simulink model "sm_Experimental_Setup"  (R2020b)
settings: Solver=VariableStepAuto  StartTime=0.0  StopTime=2000  RelTol=1e-3
values from neighbouring files (symbols this model uses):
  ACCEPTABLE_DELTA = 0.05    [code_DDPG_Training.m]    (also in code_Experimental_Setup.m; code_SA_TF_Estimator.m)
  fD = 3.5243/2    (= 1.76215)    [code_DDPG_Training.m]    (also in code_Experimental_Setup.m; code_SA_TF_Estimator.m = 3.5243)
  fS = 8.4000/2    (= 4.2)    [code_DDPG_Training.m]    (also in code_Experimental_Setup.m; code_SA_TF_Estimator.m = 8.4)
  TIME_DELAY = 2.5/2    (= 1.25)    [code_DDPG_Training.m]    (also in code_Experimental_Setup.m; code_SA_TF_Estimator.m = 2.5)
  Ts = 1.0    (= 1)    [code_DDPG_Training.m]    (also in code_Experimental_Setup.m; code_SA_TF_Estimator.m)
undefined symbols (not defined in the file or in its folder): DiscIntNeverNeededParam, sigbuilder_block
libraries: simulink x2, pid_lib x1, rllib x1
settings Model: Creator=rajeshs  LastModifiedBy=rajeshs
settings SFSimCC: CustomCodeUndefinedFunction=UseInterfaceOnly

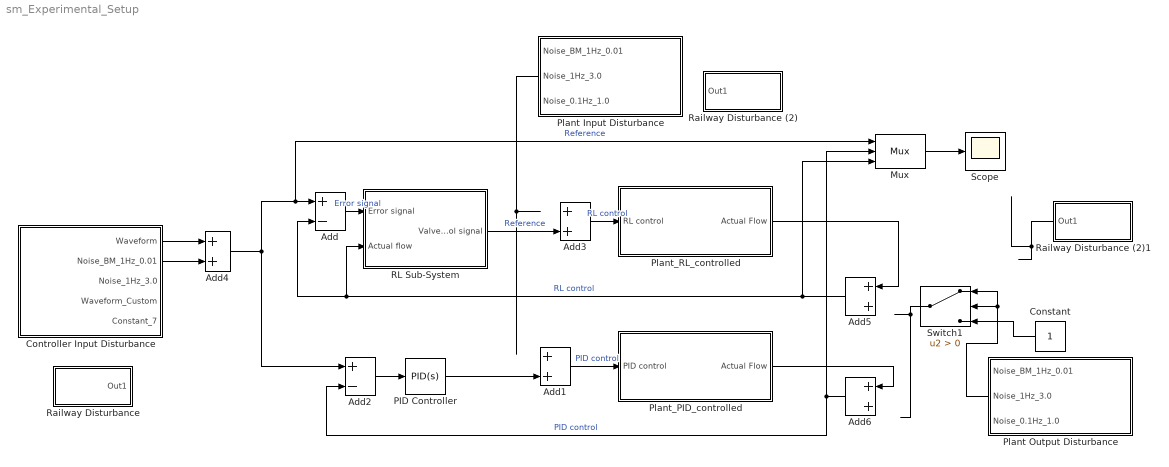
== system sm_Experimental_Setup ==
  Add : Sum  Inputs=+-
  Add{1,3..6} (5 alike) : Sum
  Add2 : Sum  Inputs=+-
  Constant : Constant
  Controller Input Disturbance : Subsystem  Tag=STV Subsys  LoadFcn=sigbuilder_block('load');  StartFcn=sigbuilder_block('start');  StopFcn=sigbuilder_block('stop');  ClipboardFcn=sigbuilder_block('clipboard');  mask(Sigbuilder block){tuvar=[0:10]}
      mask help: Simulink:masks:SigbuilderBlock_MD
      mask init:
      | if ~strcmp(get_param(bdroot(gcbh),'SimulationStatus'),'stopped') tuvar = sigbuilder_block('maskInit'); end
      settings: CopyFcn=sigbuilder_block('copy');  DeleteFcn=sigbuilder_block('delete');  ModelCloseFcn=sigbuilder_block('modelClose');  PreSaveFcn=sigbuilder_block('preSave');  PauseFcn=sigbuilder_block('pause');  ContinueFcn=sigbuilder_block('continue');  NameChangeFcn=sigbuilder_block('namechange');  OpenFcn=sigbuilder_block('open',[329.25 -26.25 324 449.25 ]);  CloseFcn=sigbuilder_block('close');
      mask Display: plot(0, 0, 100, 100,[2, 2, 32, 32, 2], [68, 8, 8, 68, 68],[32, 2], [38, 38], [32, 19, 2],[53, 60, 44], [32, 17, 17, 2],[16, 16, 31, 31]);txt = getActiveGroup(gcbh);text(2, 100, txt,'verticalAlignment', 'top');
  Mux : Mux  Inputs=3
      settings: DisplayOption=signals
  PID Controller : pid_lib/PID Controller  Controller=PID  Form=Parallel  TimeDomain=Continuous-time  UseExternalTs=off  SampleTime=-1  IntegratorMethod=Forward Euler  FilterMethod=Forward Euler  ControllerParametersSource=internal  P=0.3631  I=0.0045  D=-1.7202  UseFilter=on  N=0.0114  TunerSelectOption=Transfer Function Based (PID Tuner App)  InitialConditionSource=internal  InitialConditionForIntegrator=0  InitialConditionForFilter=0  DifferentiatorICPrevScaledInput=0  ExternalReset=none  TrackingMode=off  Kt=1  LimitOutput=off  SatLimitsSource=internal  UpperSaturationLimit=inf  LowerSaturationLimit=-inf  LinearizeAsGain=on  AntiWindupMode=none  Kb=1  POutMin=[]  POutMax=[]  IOutMin=[]  IOutMax=[]  DOutMin=[]  DOutMax=[]  NOutMin=[]  NOutMax=[]  SumOutMin=[]  SumOutMax=[]  SaturationOutMin=[]  SaturationOutMax=[]  PParamMin=[]  PParamMax=[]  IParamMin=[]  IParamMax=[]  DParamMin=[]  DParamMax=[]  NParamMin=[]  NParamMax=[]  KbParamMin=[]  KbParamMax=[]  KtParamMin=[]  KtParamMax=[]  KbOutMin=[]  KbOutMax=[]  KtOutMin=[]  KtOutMax=[]  IntegratorOutMin=[]  IntegratorOutMax=[]  FilterOutMin=[]  FilterOutMax=[]  SumI1OutMin=[]  SumI1OutMax=[]  SumI2OutMin=[]  SumI2OutMax=[]  SumI3OutMin=[]  SumI3OutMax=[]  SumI4OutMin=[]  SumI4OutMax=[]  SumDOutMin=[]  SumDOutMax=[]  DifferentiatorOutMin=[]  DifferentiatorOutMax=[]  FilterDiffOutCoefMin=[]  FilterDiffOutCoefMax=[]  ReciprocalOutMin=[]  ReciprocalOutMax=[]  SumDenOutMin=[]  SumDenOutMax=[]  SumNumOutMin=[]  SumNumOutMax=[]  DivideOutMin=[]  DivideOutMax=[]  UdiffTsProdOutMin=[]  UdiffTsProdOutMax=[]  NTsProdOutMin=[]  NTsProdOutMax=[]  UintegralTsProdOutMin=[]  UintegralTsProdOutMax=[]  UngainTsProdOutMin=[]  UngainTsProdOutMax=[]  IntegratorContinuousStateAttributes=''  IntegratorStateMustResolveToSignalObject=off  IntegratorRTWStateStorageClass=Auto  FilterContinuousStateAttributes=''  FilterStateMustResolveToSignalObject=off  FilterRTWStateStorageClass=Auto  ParallelPVariant=InternalParameters  IdealPVariant=Disabled  IVariant=InternalParameters  DVariant=InternalParameters  IntegratorVariant=Continuous  SatVariant=Disabled  AWVariant=Passthrough  PCopyVariant=Disabled  TRVariant=Disabled  FdbkBlocksVariant=Forward  IdealPFdbkVariant=Disabled  SatFdbkVariant=Disabled  DerivativeFilterVariant=ContFilter  NVariant=InternalParameters  NCopyVariant=Disabled  FilterICVariant=InternalICsFilter  IntegratorICVariant=InternalICs  ExternalResetVariant=Disabled  TRSumVariant=Passthrough  SumFdbkVariant=Disabled  SumVariant=Sum_PID  TsampFilterVariant=InternalTs  TsampNgainVariant=Passthrough  TsampIntegralVariant=Passthrough  ExternalSaturationOutDataTypeStr=Inherit: Same as second input
  Plant Input Disturbance : Subsystem  Tag=STV Subsys  LoadFcn=sigbuilder_block('load');  StartFcn=sigbuilder_block('start');  StopFcn=sigbuilder_block('stop');  ClipboardFcn=sigbuilder_block('clipboard');  mask(Sigbuilder block){tuvar=[0:10]}
      mask help: Simulink:masks:SigbuilderBlock_MD
      mask init:
      | if ~strcmp(get_param(bdroot(gcbh),'SimulationStatus'),'stopped') tuvar = sigbuilder_block('maskInit'); end
      settings: CopyFcn=sigbuilder_block('copy');  DeleteFcn=sigbuilder_block('delete');  ModelCloseFcn=sigbuilder_block('modelClose');  PreSaveFcn=sigbuilder_block('preSave');  PauseFcn=sigbuilder_block('pause');  ContinueFcn=sigbuilder_block('continue');  NameChangeFcn=sigbuilder_block('namechange');  OpenFcn=sigbuilder_block('open',[6 6 1012.5 506.25 ]);  CloseFcn=sigbuilder_block('close');
      mask Display: plot(0, 0, 100, 100,[2, 2, 32, 32, 2], [68, 8, 8, 68, 68],[32, 2], [38, 38], [32, 19, 2],[53, 60, 44], [32, 17, 17, 2],[16, 16, 31, 31]);txt = getActiveGroup(gcbh);text(2, 100, txt,'verticalAlignment', 'top');
  Plant Output Disturbance : Subsystem  Tag=STV Subsys  LoadFcn=sigbuilder_block('load');  StartFcn=sigbuilder_block('start');  StopFcn=sigbuilder_block('stop');  ClipboardFcn=sigbuilder_block('clipboard');  mask(Sigbuilder block){tuvar=[0:10]}
      mask help: Simulink:masks:SigbuilderBlock_MD
      mask init:
      | if ~strcmp(get_param(bdroot(gcbh),'SimulationStatus'),'stopped') tuvar = sigbuilder_block('maskInit'); end
      settings: CopyFcn=sigbuilder_block('copy');  DeleteFcn=sigbuilder_block('delete');  ModelCloseFcn=sigbuilder_block('modelClose');  PreSaveFcn=sigbuilder_block('preSave');  PauseFcn=sigbuilder_block('pause');  ContinueFcn=sigbuilder_block('continue');  NameChangeFcn=sigbuilder_block('namechange');  OpenFcn=sigbuilder_block('open',[6 6 1012.5 506.25 ]);  CloseFcn=sigbuilder_block('close');
      mask Display: plot(0, 0, 100, 100,[2, 2, 32, 32, 2], [68, 8, 8, 68, 68],[32, 2], [38, 38], [32, 19, 2],[53, 60, 44], [32, 17, 17, 2],[16, 16, 31, 31]);txt = getActiveGroup(gcbh);text(2, 100, txt,'verticalAlignment', 'top');
  Plant_PID_controlled : Subsystem
  Plant_RL_controlled : Subsystem
  RL Sub-System : Subsystem
  Railway Disturbance : Subsystem
  Railway Disturbance (2) : Subsystem
  Railway Disturbance (2)1 : Subsystem
  Scope : Scope
  Switch1 : Switch  Criteria=u2 > Threshold
  wires:
  Add/1 -> RL Sub-System/1(Error signal)  "Error signal"
  Add5/1 -> Mux/3, Add/2, RL Sub-System/2(Actual flow)  "RL control"
  PID Controller/1 -> Add1/2
  Add2/1 -> PID Controller/1
  Mux/1 -> Scope/1
  Add1/1 -> Plant_PID_controlled/1(PID control)  "PID control"
  Controller Input Disturbance/1(Waveform) -> Add4/1
  Add6/1 -> Mux/2, Add2/2  "PID control"
  Constant/1 -> Switch1/3
  Railway Disturbance (2)1/1(Out1) -> ?
  Switch1/1 -> ?
  Plant Input Disturbance/2(Noise_1Hz_3.0) -> ?
  Add3/1 -> Plant_RL_controlled/1(RL control)  "RL control"
  Plant_RL_controlled/1(Actual Flow) -> Add5/1
  Plant_PID_controlled/1(Actual Flow) -> Add6/1
  Controller Input Disturbance/2(Noise_BM_1Hz_0.01) -> Add4/2
  Add4/1 -> Add2/1, Mux/1, Add/1  "Reference"
  RL Sub-System/1(Valve control signal) -> Add3/2  "Reference"
  Plant Output Disturbance/2(Noise_1Hz_3.0) -> Switch1/2, Switch1/1

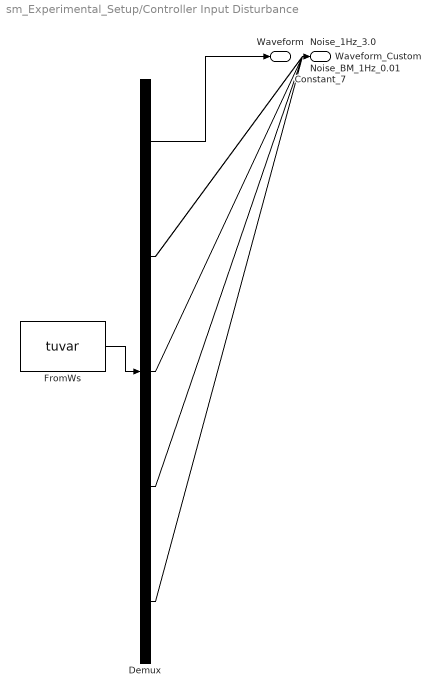
== system sm_Experimental_Setup/Controller Input Disturbance ==
  Demux : Demux  Tag=STV Demux  Outputs=5
      settings: DisplayOption=none
  FromWs : FromWorkspace  Tag=STV FromWs  VariableName=tuvar
      SigBuilderData=|
      | common.afterFinalStr = 'Extrapolate'
      | common.sampleTime = 0
      | dataSet.timeRange = [0 2000]
      | dataSet.name = 'Signals'
      | sbobj.Groups.Name = 'Signals'
      | sbobj.Groups.Signals(1).Name = 'Waveform'
      | sbobj.Groups.Signals(1).XData = [0 752 752 1500 1500 1750 1750 2000]
      | sbobj.Groups.Signals(1).YData = [100 100 25 25 75 75 25 25]
      | sbobj.Groups.Signals(2).Name = 'Noise_BM_1Hz_0.01'
      | sbobj.Groups.Signals(2).XData = [0 1 2 3 4 5 6 7 8 9 10 11 ... (2001 elements, 1x2001)]
      | sbobj.Groups.Signals(2).YData = [0.0109017282673 -0.00358703225346 -0.0012992763049 0.00733737523776 0.00120331570317 0.0113633128469 -0.00686773118719 0.00471682863443 0.00288342465456 0.0139185483505 -0.0134550201016 7.47406191734e-06 ... (2001 elements, 1x2001)]
      | sbobj.Groups.Signals(3).Name = 'Noise_1Hz_3.0'
      | sbobj.Groups.Signals(3).XData = [0 1 2 3 4 5 6 7 8 9 10 11 ... (2001 elements, 1x2001)]
      | sbobj.Groups.Signals(3).YData = [-1.22103016093 -2.32126408989 6.42034479721 -4.13028289214 0.366124868815 1.68201285192 -3.06458126709 -0.0302582378605 -4.3152453304 1.33545254952 0.451492702689 0.846422939597 ... (2001 elements, 1x2001)]
      | sbobj.Groups.Signals(4).Name = 'Waveform_Custom'
      | sbobj.Groups.Signals(4).XData = [0 100 110 200 290 398 500 600 1000 1050 1225 1400 1500 2000]
      | sbobj.Groups.Signals(4).YData = [75 75 100 100 100 20 20 75 75 10 10 100 100 5]
      | sbobj.Groups.Signals(5).Name = 'Constant_7'
      | sbobj.Groups.Signals(5).XData = [0 2000]
      | sbobj.Groups.Signals(5).YData = [100 100]
      | sbobj.Groups.TimeRange = [0 2000]
  Waveform : Outport  Tag=STV Outport  VectorParamsAs1DForOutWhenUnconnected=off
  Noise_BM_1Hz_0.01 : Outport  Tag=STV Outport  Port=2  VectorParamsAs1DForOutWhenUnconnected=off
  Noise_1Hz_3.0 : Outport  Tag=STV Outport  Port=3  VectorParamsAs1DForOutWhenUnconnected=off
  Waveform_Custom : Outport  Tag=STV Outport  Port=4  VectorParamsAs1DForOutWhenUnconnected=off
  Constant_7 : Outport  Tag=STV Outport  Port=5  VectorParamsAs1DForOutWhenUnconnected=off
  wires:
  Demux/1 -> Waveform/1
  FromWs/1 -> Demux/1
  Demux/2 -> Noise_BM_1Hz_0.01/1
  Demux/3 -> Noise_1Hz_3.0/1
  Demux/4 -> Waveform_Custom/1
  Demux/5 -> Constant_7/1

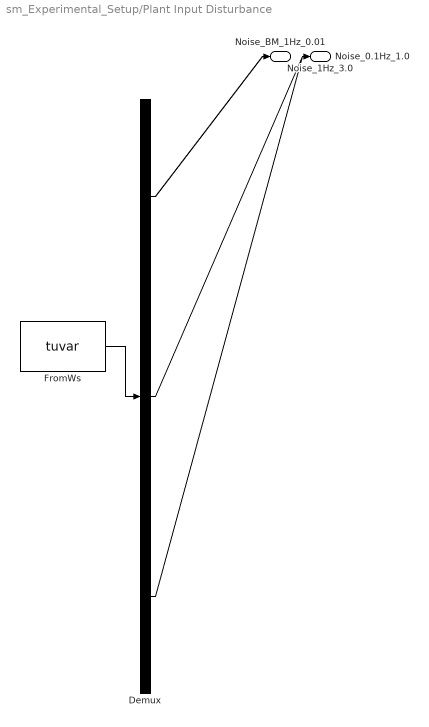
== system sm_Experimental_Setup/Plant Input Disturbance ==
  Demux : Demux  Tag=STV Demux  Outputs=3
      settings: DisplayOption=none
  FromWs : FromWorkspace  Tag=STV FromWs  VariableName=tuvar
      SigBuilderData=|
      | common.afterFinalStr = 'Extrapolate'
      | common.sampleTime = 0
      | dataSet.timeRange = [0 2000]
      | dataSet.name = 'Signals'
      | sbobj.Groups.Name = 'Signals'
      | sbobj.Groups.Signals(1).Name = 'Noise_BM_1Hz_0.01'
      | sbobj.Groups.Signals(1).XData = [0 1 2 3 4 5 6 7 8 9 10 11 ... (2001 elements, 1x2001)]
      | sbobj.Groups.Signals(1).YData = [0.0109017282673 -0.00358703225346 -0.0012992763049 0.00733737523776 0.00120331570317 0.0113633128469 -0.00686773118719 0.00471682863443 0.00288342465456 0.0139185483505 -0.0134550201016 7.47406191734e-06 ... (2001 elements, 1x2001)]
      | sbobj.Groups.Signals(2).Name = 'Noise_1Hz_3.0'
      | sbobj.Groups.Signals(2).XData = [0 1 2 3 4 5 6 7 8 9 10 11 ... (2001 elements, 1x2001)]
      | sbobj.Groups.Signals(2).YData = [-1.79047363866 1.41185835628 -7.19725460522 4.95232912088 1.68989140864 0.114208185443 0.567343325217 3.74247314685 -1.90443716599 -1.78570435989 -0.962472411073 -0.747666280685 ... (2001 elements, 1x2001)]
      | sbobj.Groups.Signals(3).Name = 'Noise_0.1Hz_1.0'
      | sbobj.Groups.Signals(3).XData = [0 10 20 30 40 50 60 70 80 90 100 110 120 130 140 150 160 170 180 190 200 210 220 230 240 250 260 270 280 290 300 310 320 330 340 350 360 370 380 390 400 410 420 430 440 450 460 470 480 490 500 510 520 530 540 550 560 570 580 590 600 610 620 630 640 650 660 670 680 690 700 710 720 730 740 750 760 770 780 790 800 810 820 830 840 850 860 870 880 890 900 910 920 930 940 950 960 970 980 990 1000 1010 1020 1030 1040 1050 1060 1070 1080 1090 1100 1110 1120 1130 1140 1150 1160 1170 1180 1190 1200 1210 1220 1230 1240 1250 1260 1270 1280 1290 1300 1310 1320 1330 1340 1350 1360 1370 1380 1390 1400 1410 1420 1430 1440 1450 1460 1470 1480 1490 1500 1510 1520 1530 1540 1550 1560 1570 1580 1590 1600 1610 1620 1630 1640 1650 1660 1670 1680 1690 1700 1710 1720 1730 1740 1750 1760 1770 1780 1790 1800 1810 1820 1830 1840 1850 1860 1870 1880 1890 1900 1910 1920 1930 1940 1950 1960 1970 1980 1990 2000]
      | sbobj.Groups.Signals(3).YData = [-0.897770229062 -1.24409162366 -0.169459534439 0.984418939663 -0.25104223595 -0.783659850186 0.308330648127 0.156728181712 0.673558474636 0.532804033794 2.10675302476 -1.10578974409 ... (201 elements, 1x201)]
      | sbobj.Groups.TimeRange = [0 2000]
  Noise_BM_1Hz_0.01 : Outport  Tag=STV Outport  VectorParamsAs1DForOutWhenUnconnected=off
  Noise_1Hz_3.0 : Outport  Tag=STV Outport  Port=2  VectorParamsAs1DForOutWhenUnconnected=off
  Noise_0.1Hz_1.0 : Outport  Tag=STV Outport  Port=3  VectorParamsAs1DForOutWhenUnconnected=off
  wires:
  FromWs/1 -> Demux/1
  Demux/1 -> Noise_BM_1Hz_0.01/1
  Demux/2 -> Noise_1Hz_3.0/1
  Demux/3 -> Noise_0.1Hz_1.0/1

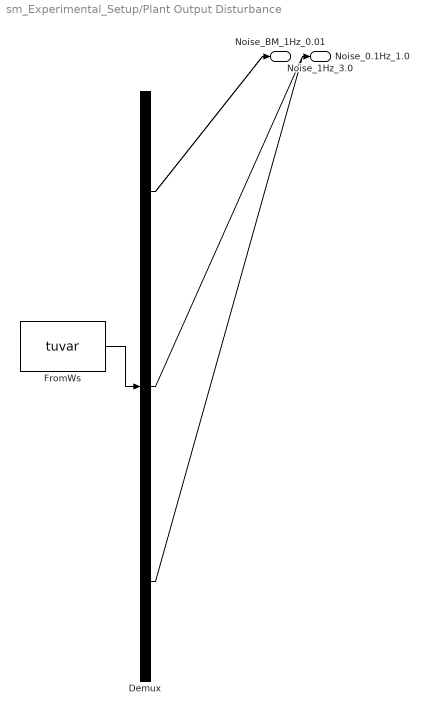
== system sm_Experimental_Setup/Plant Output Disturbance ==
  Demux : Demux  Tag=STV Demux  Outputs=3
      settings: DisplayOption=none
  FromWs : FromWorkspace  Tag=STV FromWs  VariableName=tuvar
      SigBuilderData=|
      | common.afterFinalStr = 'Extrapolate'
      | common.sampleTime = 0
      | dataSet.timeRange = [0 2000]
      | dataSet.name = 'Signals'
      | sbobj.Groups.Name = 'Signals'
      | sbobj.Groups.Signals(1).Name = 'Noise_BM_1Hz_0.01'
      | sbobj.Groups.Signals(1).XData = [0 1 2 3 4 5 6 7 8 9 10 11 ... (2001 elements, 1x2001)]
      | sbobj.Groups.Signals(1).YData = [0.0109017282673 -0.00358703225346 -0.0012992763049 0.00733737523776 0.00120331570317 0.0113633128469 -0.00686773118719 0.00471682863443 0.00288342465456 0.0139185483505 -0.0134550201016 7.47406191734e-06 ... (2001 elements, 1x2001)]
      | sbobj.Groups.Signals(2).Name = 'Noise_1Hz_3.0'
      | sbobj.Groups.Signals(2).XData = [0 1 2 3 4 5 6 7 8 9 10 11 ... (2001 elements, 1x2001)]
      | sbobj.Groups.Signals(2).YData = [-1.22103016093 -2.32126408989 6.42034479721 -4.13028289214 0.366124868815 1.68201285192 -3.06458126709 -0.0302582378605 -4.3152453304 1.33545254952 0.451492702689 0.846422939597 ... (2001 elements, 1x2001)]
      | sbobj.Groups.Signals(3).Name = 'Noise_0.1Hz_1.0'
      | sbobj.Groups.Signals(3).XData = [0 10 20 30 40 50 60 70 80 90 100 110 120 130 140 150 160 170 180 190 200 210 220 230 240 250 260 270 280 290 300 310 320 330 340 350 360 370 380 390 400 410 420 430 440 450 460 470 480 490 500 510 520 530 540 550 560 570 580 590 600 610 620 630 640 650 660 670 680 690 700 710 720 730 740 750 760 770 780 790 800 810 820 830 840 850 860 870 880 890 900 910 920 930 940 950 960 970 980 990 1000 1010 1020 1030 1040 1050 1060 1070 1080 1090 1100 1110 1120 1130 1140 1150 1160 1170 1180 1190 1200 1210 1220 1230 1240 1250 1260 1270 1280 1290 1300 1310 1320 1330 1340 1350 1360 1370 1380 1390 1400 1410 1420 1430 1440 1450 1460 1470 1480 1490 1500 1510 1520 1530 1540 1550 1560 1570 1580 1590 1600 1610 1620 1630 1640 1650 1660 1670 1680 1690 1700 1710 1720 1730 1740 1750 1760 1770 1780 1790 1800 1810 1820 1830 1840 1850 1860 1870 1880 1890 1900 1910 1920 1930 1940 1950 1960 1970 1980 1990 2000]
      | sbobj.Groups.Signals(3).YData = [-0.897770229062 -1.24409162366 -0.169459534439 0.984418939663 -0.25104223595 -0.783659850186 0.308330648127 0.156728181712 0.673558474636 0.532804033794 2.10675302476 -1.10578974409 ... (201 elements, 1x201)]
      | sbobj.Groups.TimeRange = [0 2000]
  Noise_BM_1Hz_0.01 : Outport  Tag=STV Outport  VectorParamsAs1DForOutWhenUnconnected=off
  Noise_1Hz_3.0 : Outport  Tag=STV Outport  Port=2  VectorParamsAs1DForOutWhenUnconnected=off
  Noise_0.1Hz_1.0 : Outport  Tag=STV Outport  Port=3  VectorParamsAs1DForOutWhenUnconnected=off
  wires:
  FromWs/1 -> Demux/1
  Demux/1 -> Noise_BM_1Hz_0.01/1
  Demux/2 -> Noise_1Hz_3.0/1
  Demux/3 -> Noise_0.1Hz_1.0/1

== system sm_Experimental_Setup/Plant_PID_controlled ==
  PID control : Inport
  Non-linear Valve model : Subsystem
  Process : Subsystem
  Actual Flow : Outport  VectorParamsAs1DForOutWhenUnconnected=off
  wires:
  Non-linear Valve model/1(ValveOutput) -> Process/1(Valve control)
  Process/1(Controlled_Flow) -> Actual Flow/1  "Actual Flow"
  PID control/1 -> Non-linear Valve model/1(ValveInput)

== system sm_Experimental_Setup/Plant_RL_controlled ==
  RL control : Inport
  Non-linear Valve model : Subsystem
  Process : Subsystem
  Actual Flow : Outport  VectorParamsAs1DForOutWhenUnconnected=off
  wires:
  Non-linear Valve model/1(ValveOutput) -> Process/1(Valve control)
  Process/1(Controlled_Flow) -> Actual Flow/1  "Actual Flow"
  RL control/1 -> Non-linear Valve model/1(ValveInput)

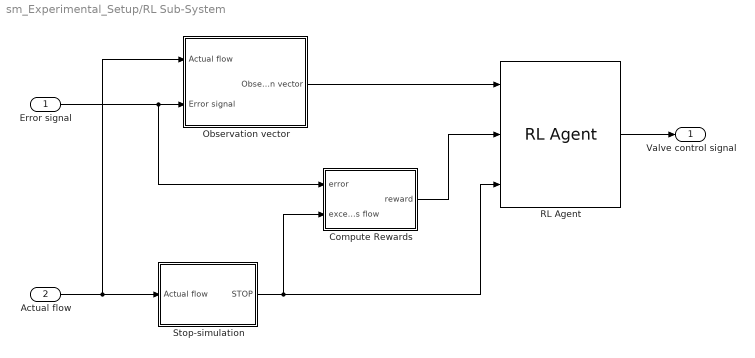
== system sm_Experimental_Setup/RL Sub-System ==
  Error signal : Inport
  Actual flow : Inport  Port=2
  Compute Rewards : Subsystem
  Observation vector : Subsystem
  RL Agent : rllib/RL Agent  Agent=agent  ProvideReward=on  ProvideIsDone=on  ProvideCumRwd=off  TreatAsDirectFeedthrough=on  CollectLoggedSignals=on  CollectModelStates=on
  Stop-simulation : Subsystem
  Valve control signal : Outport  VectorParamsAs1DForOutWhenUnconnected=off
  wires:
  Stop-simulation/1(STOP) -> RL Agent/3, Compute Rewards/2(exceeds flow)
  Error signal/1 -> Compute Rewards/1(error), Observation vector/2(Error signal)
  Compute Rewards/1(reward) -> RL Agent/2
  Observation vector/1(Observation vector) -> RL Agent/1
  RL Agent/1 -> Valve control signal/1
  Actual flow/1 -> Observation vector/1(Actual flow), Stop-simulation/1(Actual flow)

== system sm_Experimental_Setup/Railway Disturbance ==
  Add7 : Sum  Inputs=3
  "RailwayDisturbance " : Subsystem  Tag=STV Subsys  LoadFcn=sigbuilder_block('load');  StartFcn=sigbuilder_block('start');  StopFcn=sigbuilder_block('stop');  ClipboardFcn=sigbuilder_block('clipboard');  mask(Sigbuilder block){tuvar=[0:10]}
      mask help: Simulink:masks:SigbuilderBlock_MD
      mask init:
      | if ~strcmp(get_param(bdroot(gcbh),'SimulationStatus'),'stopped') tuvar = sigbuilder_block('maskInit'); end
      settings: CopyFcn=sigbuilder_block('copy');  DeleteFcn=sigbuilder_block('delete');  ModelCloseFcn=sigbuilder_block('modelClose');  PreSaveFcn=sigbuilder_block('preSave');  PauseFcn=sigbuilder_block('pause');  ContinueFcn=sigbuilder_block('continue');  NameChangeFcn=sigbuilder_block('namechange');  OpenFcn=sigbuilder_block('open',[401.25 -15.75 441 506.25 ]);  CloseFcn=sigbuilder_block('close');
      mask Display: plot(0, 0, 100, 100,[2, 2, 32, 32, 2], [68, 8, 8, 68, 68],[32, 2], [38, 38], [32, 19, 2],[53, 60, 44], [32, 17, 17, 2],[16, 16, 31, 31]);txt = getActiveGroup(gcbh);text(2, 100, txt,'verticalAlignment', 'top');
  Out1 : Outport  VectorParamsAs1DForOutWhenUnconnected=off
  wires:
  "RailwayDisturbance "/3(RW_1.0_1.0) -> Add7/3
  Add7/1 -> Out1/1
  "RailwayDisturbance "/1(RW_50_1.0) -> Add7/1
  "RailwayDisturbance "/2(RW_0.01_3.0) -> Add7/2

== system sm_Experimental_Setup/Railway Disturbance (2) ==
  Add7 : Sum  Inputs=3
  "RailwayDisturbance " : Subsystem  Tag=STV Subsys  LoadFcn=sigbuilder_block('load');  StartFcn=sigbuilder_block('start');  StopFcn=sigbuilder_block('stop');  ClipboardFcn=sigbuilder_block('clipboard');  mask(Sigbuilder block){tuvar=[0:10]}
      mask help: Simulink:masks:SigbuilderBlock_MD
      mask init:
      | if ~strcmp(get_param(bdroot(gcbh),'SimulationStatus'),'stopped') tuvar = sigbuilder_block('maskInit'); end
      settings: CopyFcn=sigbuilder_block('copy');  DeleteFcn=sigbuilder_block('delete');  ModelCloseFcn=sigbuilder_block('modelClose');  PreSaveFcn=sigbuilder_block('preSave');  PauseFcn=sigbuilder_block('pause');  ContinueFcn=sigbuilder_block('continue');  NameChangeFcn=sigbuilder_block('namechange');  OpenFcn=sigbuilder_block('open',[577.5 6 441 506.25 ]);  CloseFcn=sigbuilder_block('close');
      mask Display: plot(0, 0, 100, 100,[2, 2, 32, 32, 2], [68, 8, 8, 68, 68],[32, 2], [38, 38], [32, 19, 2],[53, 60, 44], [32, 17, 17, 2],[16, 16, 31, 31]);txt = getActiveGroup(gcbh);text(2, 100, txt,'verticalAlignment', 'top');
  Out1 : Outport  VectorParamsAs1DForOutWhenUnconnected=off
  wires:
  "RailwayDisturbance "/3(RW_1.0_1.0) -> Add7/3
  Add7/1 -> Out1/1
  "RailwayDisturbance "/1(RW_50_1.0) -> Add7/1
  "RailwayDisturbance "/2(RW_0.01_3.0) -> Add7/2

== system sm_Experimental_Setup/Railway Disturbance (2)1 ==
  Add7 : Sum  Inputs=3
  "RailwayDisturbance " : Subsystem  Tag=STV Subsys  LoadFcn=sigbuilder_block('load');  StartFcn=sigbuilder_block('start');  StopFcn=sigbuilder_block('stop');  ClipboardFcn=sigbuilder_block('clipboard');  mask(Sigbuilder block){tuvar=[0:10]}
      mask help: Simulink:masks:SigbuilderBlock_MD
      mask init:
      | if ~strcmp(get_param(bdroot(gcbh),'SimulationStatus'),'stopped') tuvar = sigbuilder_block('maskInit'); end
      settings: CopyFcn=sigbuilder_block('copy');  DeleteFcn=sigbuilder_block('delete');  ModelCloseFcn=sigbuilder_block('modelClose');  PreSaveFcn=sigbuilder_block('preSave');  PauseFcn=sigbuilder_block('pause');  ContinueFcn=sigbuilder_block('continue');  NameChangeFcn=sigbuilder_block('namechange');  OpenFcn=sigbuilder_block('open',[577.5 6 441 506.25 ]);  CloseFcn=sigbuilder_block('close');
      mask Display: plot(0, 0, 100, 100,[2, 2, 32, 32, 2], [68, 8, 8, 68, 68],[32, 2], [38, 38], [32, 19, 2],[53, 60, 44], [32, 17, 17, 2],[16, 16, 31, 31]);txt = getActiveGroup(gcbh);text(2, 100, txt,'verticalAlignment', 'top');
  Out1 : Outport  VectorParamsAs1DForOutWhenUnconnected=off
  wires:
  "RailwayDisturbance "/3(RW_1.0_1.0) -> Add7/3
  Add7/1 -> Out1/1
  "RailwayDisturbance "/1(RW_50_1.0) -> Add7/1
  "RailwayDisturbance "/2(RW_0.01_3.0) -> Add7/2

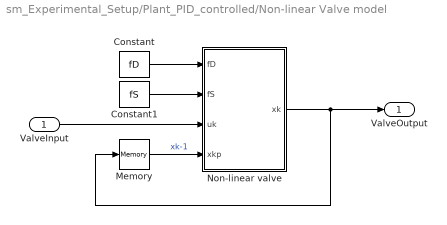
== system sm_Experimental_Setup/Plant_PID_controlled/Non-linear Valve model ==
  ValveInput : Inport
  Constant : Constant  Value=fD
  Constant1 : Constant  Value=fS
  Memory : Memory
  Non-linear valve : MATLAB Function  TreatAsAtomicUnit=on
  ValveOutput : Outport  VectorParamsAs1DForOutWhenUnconnected=off
  wires:
  Non-linear valve/1(xk) -> ValveOutput/1, Memory/1
  Memory/1 -> Non-linear valve/4(xkp)  "xk-1"
  ValveInput/1 -> Non-linear valve/3(uk)
  Constant/1 -> Non-linear valve/1(fD)
  Constant1/1 -> Non-linear valve/2(fS)

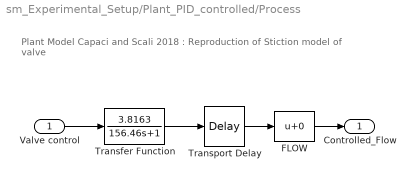
== system sm_Experimental_Setup/Plant_PID_controlled/Process ==
  note: Plant Model
      |
      | Capaci and Scali 2018 : Reproduction of Stiction model of valve
  Valve control : Inport
  FLOW : Bias
  Transfer Function : TransferFcn  Numerator=[3.8163]  Denominator=[156.46 1]
  "Transport Delay " : TransportDelay  DelayTime=TIME_DELAY
  Controlled_Flow : Outport  VectorParamsAs1DForOutWhenUnconnected=off
  wires:
  FLOW/1 -> Controlled_Flow/1
  Transfer Function/1 -> "Transport Delay "/1
  Valve control/1 -> Transfer Function/1
  "Transport Delay "/1 -> FLOW/1

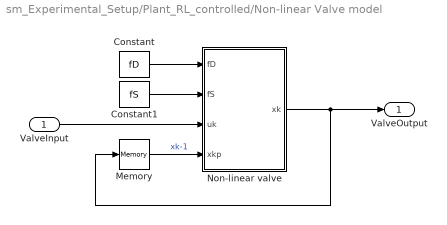
== system sm_Experimental_Setup/Plant_RL_controlled/Non-linear Valve model ==
  ValveInput : Inport
  Constant : Constant  Value=fD
  Constant1 : Constant  Value=fS
  Memory : Memory
  Non-linear valve : MATLAB Function  TreatAsAtomicUnit=on
  ValveOutput : Outport  VectorParamsAs1DForOutWhenUnconnected=off
  wires:
  Non-linear valve/1(xk) -> ValveOutput/1, Memory/1
  Memory/1 -> Non-linear valve/4(xkp)  "xk-1"
  ValveInput/1 -> Non-linear valve/3(uk)
  Constant/1 -> Non-linear valve/1(fD)
  Constant1/1 -> Non-linear valve/2(fS)

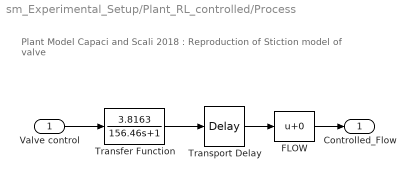
== system sm_Experimental_Setup/Plant_RL_controlled/Process ==
  note: Plant Model
      |
      | Capaci and Scali 2018 : Reproduction of Stiction model of valve
  Valve control : Inport
  FLOW : Bias
  Transfer Function : TransferFcn  Numerator=[3.8163]  Denominator=[156.46 1]
  "Transport Delay " : TransportDelay  DelayTime=TIME_DELAY
  Controlled_Flow : Outport  VectorParamsAs1DForOutWhenUnconnected=off
  wires:
  FLOW/1 -> Controlled_Flow/1
  Transfer Function/1 -> "Transport Delay "/1
  Valve control/1 -> Transfer Function/1
  "Transport Delay "/1 -> FLOW/1

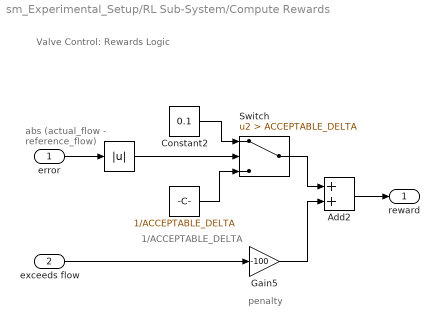
== system sm_Experimental_Setup/RL Sub-System/Compute Rewards ==
  note: penalty
  note: 1/ACCEPTABLE_DELTA
  note: abs (actual_flow - reference_flow)
  note: Valve Control: Rewards Logic
  error : Inport
  exceeds flow : Inport  Port=2
  " " : Constant  Value=1/ACCEPTABLE_DELTA
  " " : Abs
  Add2 : Sum
  Constant2 : Constant  Value=0.1
  Gain5 : Gain  Gain=-100
  Switch : Switch  Criteria=u2 > Threshold  Threshold=ACCEPTABLE_DELTA
  reward : Outport  VectorParamsAs1DForOutWhenUnconnected=off
  wires:
  Gain5/1 -> Add2/2
  exceeds flow/1 -> Gain5/1
  error/1 -> " "/1
  Add2/1 -> reward/1
  " "/1 -> Switch/2
  " "/1 -> Switch/3
  Constant2/1 -> Switch/1
  Switch/1 -> Add2/1

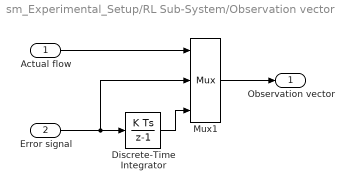
== system sm_Experimental_Setup/RL Sub-System/Observation vector ==
  Actual flow : Inport
  Error signal : Inport  Port=2
  Discrete-Time Integrator : DiscreteIntegrator  SampleTime=Ts  ICPrevOutput=DiscIntNeverNeededParam  ICPrevScaledInput=DiscIntNeverNeededParam
  Mux1 : Mux  Inputs=3
  Observation vector : Outport  VectorParamsAs1DForOutWhenUnconnected=off
  wires:
  Discrete-Time Integrator/1 -> Mux1/3
  Mux1/1 -> Observation vector/1
  Error signal/1 -> Discrete-Time Integrator/1, Mux1/2
  Actual flow/1 -> Mux1/1

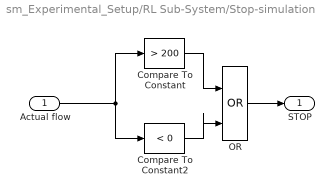
== system sm_Experimental_Setup/RL Sub-System/Stop-simulation ==
  Actual flow : Inport
  Compare To Constant : simulink/Logic and Bit Operations/Compare To Constant  relop=>  const=200  OutDataTypeStr=boolean
  Compare To Constant2 : simulink/Logic and Bit Operations/Compare To Constant  relop=<  const=0  OutDataTypeStr=boolean
  OR : Logic  Operator=OR  IconShape=distinctive  AllPortsSameDT=off  OutDataTypeStr=boolean
  STOP : Outport  VectorParamsAs1DForOutWhenUnconnected=off
  wires:
  Compare To Constant/1 -> OR/1
  Actual flow/1 -> Compare To Constant/1, Compare To Constant2/1
  Compare To Constant2/1 -> OR/2
  OR/1 -> STOP/1

== system sm_Experimental_Setup/Railway Disturbance/RailwayDisturbance  ==
  Demux : Demux  Tag=STV Demux  Outputs=3
      settings: DisplayOption=none
  FromWs : FromWorkspace  Tag=STV FromWs  VariableName=tuvar
      SigBuilderData=|
      | common.afterFinalStr = 'Extrapolate'
      | common.sampleTime = 0
      | dataSet(1).timeRange = [0 2000]
      | dataSet(1).name = 'Signals'
      | dataSet(2).timeRange = [0 2000]
      | dataSet(2).name = 'Signals1'
      | sbobj.Groups(1).Name = 'Signals'
      | sbobj.Groups(1).Signals(1).Name = 'RW_50_1.0'
      | sbobj.Groups(1).Signals(1).XData = [0 0.01 0.02 0.03 0.04 0.05 0.06 0.07 0.08 0.09 0.1 0.11 ... (200001 elements, 1x200001)]
      | sbobj.Groups(1).Signals(1).YData = [0.0748964902718 -0.290373671365 -2.35413855295 -0.25683543375 0.827171869303 0.735199489712 -0.389698055073 1.41120657442 0.386602820528 0.310514016169 0.550562819733 0.141974999783 ... (200001 elements, 1x200001)]
      | sbobj.Groups(1).Signals(2).Name = 'RW_0.01_3.0'
      | sbobj.Groups(1).Signals(2).XData = [0 100 200 300 400 500 600 700 800 900 1000 1100 1200 1300 1400 1500 1600 1700 1800 1900 2000]
      | sbobj.Groups(1).Signals(2).YData = [-1.75041208804 5.00208214186 -0.81766709166 -1.72755502884 -3.19474663133 -2.29477094753 -0.864480416247 -2.28910225428 2.52055988421 -0.221233052931 4.2711123865 -1.03334701442 -1.36012274107 -0.824925329157 -6.62107730698 -3.81352548468 -0.295571577622 -5.39720756813 -1.49875789598 4.16778533923 0.957257557404]
      | sbobj.Groups(1).Signals(3).Name = 'RW_1.0_1.0'
      | sbobj.Groups(1).Signals(3).XData = [0 1 2 3 4 5 6 7 8 9 10 11 ... (2001 elements, 1x2001)]
      | sbobj.Groups(1).Signals(3).YData = [-0.784346883609 0.62301436161 -1.51105459971 -1.26389181978 0.298467304534 0.219842773188 1.17100891999 -0.898884099641 0.0733312203911 0.421761490034 0.70336183435 1.19088493109 ... (2001 elements, 1x2001)]
      | sbobj.Groups(1).TimeRange = [0 2000]
      | sbobj.Groups(2).Name = 'Signals1'
      | sbobj.Groups(2).Signals(1).Name = 'RW_50_1.0'
      | sbobj.Groups(2).Signals(1).XData = [0 0.02 0.04 0.06 0.08 0.1 0.12 0.14 0.16 0.18 0.2 0.22 ... (100001 elements, 1x100001)]
      | sbobj.Groups(2).Signals(1).YData = [0.848186559425 -1.5008078928 -0.621890626664 -1.2492106404 2.4723414477 0.929972259963 1.13942527491 -1.26800419674 -0.133921777363 -0.0585727313123 0.553050501105 0.425683651949 ... (100001 elements, 1x100001)]
      | sbobj.Groups(2).Signals(2).Name = 'RW_0.01_3.0'
      | sbobj.Groups(2).Signals(2).XData = [0 100 200 300 400 500 600 700 800 900 1000 1100 1200 1300 1400 1500 1600 1700 1800 1900 2000]
      | sbobj.Groups(2).Signals(2).YData = [-1.75041208804 5.00208214186 -0.81766709166 -1.72755502884 -3.19474663133 -2.29477094753 -0.864480416247 -2.28910225428 2.52055988421 -0.221233052931 4.2711123865 -1.03334701442 -1.36012274107 -0.824925329157 -6.62107730698 -3.81352548468 -0.295571577622 -5.39720756813 -1.49875789598 4.16778533923 0.957257557404]
      | sbobj.Groups(2).Signals(3).Name = 'RW_1.0_1.0'
      | sbobj.Groups(2).Signals(3).XData = [0 1 2 3 4 5 6 7 8 9 10 11 ... (2001 elements, 1x2001)]
      | sbobj.Groups(2).Signals(3).YData = [-0.784346883609 0.62301436161 -1.51105459971 -1.26389181978 0.298467304534 0.219842773188 1.17100891999 -0.898884099641 0.0733312203911 0.421761490034 0.70336183435 1.19088493109 ... (2001 elements, 1x2001)]
      | sbobj.Groups(2).TimeRange = [0 2000]
  RW_50_1.0 : Outport  Tag=STV Outport  VectorParamsAs1DForOutWhenUnconnected=off
  RW_0.01_3.0 : Outport  Tag=STV Outport  Port=2  VectorParamsAs1DForOutWhenUnconnected=off
  RW_1.0_1.0 : Outport  Tag=STV Outport  Port=3  VectorParamsAs1DForOutWhenUnconnected=off
  wires:
  FromWs/1 -> Demux/1
  Demux/1 -> RW_50_1.0/1
  Demux/2 -> RW_0.01_3.0/1
  Demux/3 -> RW_1.0_1.0/1

== system sm_Experimental_Setup/Railway Disturbance (2)/RailwayDisturbance  ==
  Demux : Demux  Tag=STV Demux  Outputs=3
      settings: DisplayOption=none
  FromWs : FromWorkspace  Tag=STV FromWs  VariableName=tuvar
      SigBuilderData=|
      | common.afterFinalStr = 'Extrapolate'
      | common.sampleTime = 0
      | dataSet(1).timeRange = [0 2000]
      | dataSet(1).name = 'Signals'
      | dataSet(2).timeRange = [0 2000]
      | dataSet(2).name = 'Signals1'
      | sbobj.Groups(1).Name = 'Signals'
      | sbobj.Groups(1).Signals(1).Name = 'RW_50_1.0'
      | sbobj.Groups(1).Signals(1).XData = [0 0.02 0.04 0.06 0.08 0.1 0.12 0.14 0.16 0.18 0.2 0.22 ... (100001 elements, 1x100001)]
      | sbobj.Groups(1).Signals(1).YData = [0.848186559425 -1.5008078928 -0.621890626664 -1.2492106404 2.4723414477 0.929972259963 1.13942527491 -1.26800419674 -0.133921777363 -0.0585727313123 0.553050501105 0.425683651949 ... (100001 elements, 1x100001)]
      | sbobj.Groups(1).Signals(2).Name = 'RW_0.01_3.0'
      | sbobj.Groups(1).Signals(2).XData = [0 100 200 300 400 500 600 700 800 900 1000 1100 1200 1300 1400 1500 1600 1700 1800 1900 2000]
      | sbobj.Groups(1).Signals(2).YData = [-1.75041208804 5.00208214186 -0.81766709166 -1.72755502884 -3.19474663133 -2.29477094753 -0.864480416247 -2.28910225428 2.52055988421 -0.221233052931 4.2711123865 -1.03334701442 -1.36012274107 -0.824925329157 -6.62107730698 -3.81352548468 -0.295571577622 -5.39720756813 -1.49875789598 4.16778533923 0.957257557404]
      | sbobj.Groups(1).Signals(3).Name = 'RW_1.0_1.0'
      | sbobj.Groups(1).Signals(3).XData = [0 1 2 3 4 5 6 7 8 9 10 11 ... (2001 elements, 1x2001)]
      | sbobj.Groups(1).Signals(3).YData = [-0.784346883609 0.62301436161 -1.51105459971 -1.26389181978 0.298467304534 0.219842773188 1.17100891999 -0.898884099641 0.0733312203911 0.421761490034 0.70336183435 1.19088493109 ... (2001 elements, 1x2001)]
      | sbobj.Groups(1).TimeRange = [0 2000]
      | sbobj.Groups(2).Name = 'Signals1'
      | sbobj.Groups(2).Signals(1).Name = 'RW_50_1.0'
      | sbobj.Groups(2).Signals(1).XData = [0 0.02 0.04 0.06 0.08 0.1 0.12 0.14 0.16 0.18 0.2 0.22 ... (100001 elements, 1x100001)]
      | sbobj.Groups(2).Signals(1).YData = [0.848186559425 -1.5008078928 -0.621890626664 -1.2492106404 2.4723414477 0.929972259963 1.13942527491 -1.26800419674 -0.133921777363 -0.0585727313123 0.553050501105 0.425683651949 ... (100001 elements, 1x100001)]
      | sbobj.Groups(2).Signals(2).Name = 'RW_0.01_3.0'
      | sbobj.Groups(2).Signals(2).XData = [0 100 200 300 400 500 600 700 800 900 1000 1100 1200 1300 1400 1500 1600 1700 1800 1900 2000]
      | sbobj.Groups(2).Signals(2).YData = [-1.75041208804 5.00208214186 -0.81766709166 -1.72755502884 -3.19474663133 -2.29477094753 -0.864480416247 -2.28910225428 2.52055988421 -0.221233052931 4.2711123865 -1.03334701442 -1.36012274107 -0.824925329157 -6.62107730698 -3.81352548468 -0.295571577622 -5.39720756813 -1.49875789598 4.16778533923 0.957257557404]
      | sbobj.Groups(2).Signals(3).Name = 'RW_1.0_1.0'
      | sbobj.Groups(2).Signals(3).XData = [0 1 2 3 4 5 6 7 8 9 10 11 ... (2001 elements, 1x2001)]
      | sbobj.Groups(2).Signals(3).YData = [-0.784346883609 0.62301436161 -1.51105459971 -1.26389181978 0.298467304534 0.219842773188 1.17100891999 -0.898884099641 0.0733312203911 0.421761490034 0.70336183435 1.19088493109 ... (2001 elements, 1x2001)]
      | sbobj.Groups(2).TimeRange = [0 2000]
  RW_50_1.0 : Outport  Tag=STV Outport  VectorParamsAs1DForOutWhenUnconnected=off
  RW_0.01_3.0 : Outport  Tag=STV Outport  Port=2  VectorParamsAs1DForOutWhenUnconnected=off
  RW_1.0_1.0 : Outport  Tag=STV Outport  Port=3  VectorParamsAs1DForOutWhenUnconnected=off
  wires:
  FromWs/1 -> Demux/1
  Demux/1 -> RW_50_1.0/1
  Demux/2 -> RW_0.01_3.0/1
  Demux/3 -> RW_1.0_1.0/1

== system sm_Experimental_Setup/Railway Disturbance (2)1/RailwayDisturbance  ==
  Demux : Demux  Tag=STV Demux  Outputs=3
      settings: DisplayOption=none
  FromWs : FromWorkspace  Tag=STV FromWs  VariableName=tuvar
      SigBuilderData=|
      | common.afterFinalStr = 'Extrapolate'
      | common.sampleTime = 0
      | dataSet(1).timeRange = [0 2000]
      | dataSet(1).name = 'Signals'
      | dataSet(2).timeRange = [0 2000]
      | dataSet(2).name = 'Signals1'
      | sbobj.Groups(1).Name = 'Signals'
      | sbobj.Groups(1).Signals(1).Name = 'RW_50_1.0'
      | sbobj.Groups(1).Signals(1).XData = [0 0.02 0.04 0.06 0.08 0.1 0.12 0.14 0.16 0.18 0.2 0.22 ... (100001 elements, 1x100001)]
      | sbobj.Groups(1).Signals(1).YData = [0.848186559425 -1.5008078928 -0.621890626664 -1.2492106404 2.4723414477 0.929972259963 1.13942527491 -1.26800419674 -0.133921777363 -0.0585727313123 0.553050501105 0.425683651949 ... (100001 elements, 1x100001)]
      | sbobj.Groups(1).Signals(2).Name = 'RW_0.01_3.0'
      | sbobj.Groups(1).Signals(2).XData = [0 100 200 300 400 500 600 700 800 900 1000 1100 1200 1300 1400 1500 1600 1700 1800 1900 2000]
      | sbobj.Groups(1).Signals(2).YData = [-1.75041208804 5.00208214186 -0.81766709166 -1.72755502884 -3.19474663133 -2.29477094753 -0.864480416247 -2.28910225428 2.52055988421 -0.221233052931 4.2711123865 -1.03334701442 -1.36012274107 -0.824925329157 -6.62107730698 -3.81352548468 -0.295571577622 -5.39720756813 -1.49875789598 4.16778533923 0.957257557404]
      | sbobj.Groups(1).Signals(3).Name = 'RW_1.0_1.0'
      | sbobj.Groups(1).Signals(3).XData = [0 1 2 3 4 5 6 7 8 9 10 11 ... (2001 elements, 1x2001)]
      | sbobj.Groups(1).Signals(3).YData = [-0.784346883609 0.62301436161 -1.51105459971 -1.26389181978 0.298467304534 0.219842773188 1.17100891999 -0.898884099641 0.0733312203911 0.421761490034 0.70336183435 1.19088493109 ... (2001 elements, 1x2001)]
      | sbobj.Groups(1).TimeRange = [0 2000]
      | sbobj.Groups(2).Name = 'Signals1'
      | sbobj.Groups(2).Signals(1).Name = 'RW_50_1.0'
      | sbobj.Groups(2).Signals(1).XData = [0 0.02 0.04 0.06 0.08 0.1 0.12 0.14 0.16 0.18 0.2 0.22 ... (100001 elements, 1x100001)]
      | sbobj.Groups(2).Signals(1).YData = [0.848186559425 -1.5008078928 -0.621890626664 -1.2492106404 2.4723414477 0.929972259963 1.13942527491 -1.26800419674 -0.133921777363 -0.0585727313123 0.553050501105 0.425683651949 ... (100001 elements, 1x100001)]
      | sbobj.Groups(2).Signals(2).Name = 'RW_0.01_3.0'
      | sbobj.Groups(2).Signals(2).XData = [0 100 200 300 400 500 600 700 800 900 1000 1100 1200 1300 1400 1500 1600 1700 1800 1900 2000]
      | sbobj.Groups(2).Signals(2).YData = [-1.75041208804 5.00208214186 -0.81766709166 -1.72755502884 -3.19474663133 -2.29477094753 -0.864480416247 -2.28910225428 2.52055988421 -0.221233052931 4.2711123865 -1.03334701442 -1.36012274107 -0.824925329157 -6.62107730698 -3.81352548468 -0.295571577622 -5.39720756813 -1.49875789598 4.16778533923 0.957257557404]
      | sbobj.Groups(2).Signals(3).Name = 'RW_1.0_1.0'
      | sbobj.Groups(2).Signals(3).XData = [0 1 2 3 4 5 6 7 8 9 10 11 ... (2001 elements, 1x2001)]
      | sbobj.Groups(2).Signals(3).YData = [-0.784346883609 0.62301436161 -1.51105459971 -1.26389181978 0.298467304534 0.219842773188 1.17100891999 -0.898884099641 0.0733312203911 0.421761490034 0.70336183435 1.19088493109 ... (2001 elements, 1x2001)]
      | sbobj.Groups(2).TimeRange = [0 2000]
  RW_50_1.0 : Outport  Tag=STV Outport  VectorParamsAs1DForOutWhenUnconnected=off
  RW_0.01_3.0 : Outport  Tag=STV Outport  Port=2  VectorParamsAs1DForOutWhenUnconnected=off
  RW_1.0_1.0 : Outport  Tag=STV Outport  Port=3  VectorParamsAs1DForOutWhenUnconnected=off
  wires:
  FromWs/1 -> Demux/1
  Demux/1 -> RW_50_1.0/1
  Demux/2 -> RW_0.01_3.0/1
  Demux/3 -> RW_1.0_1.0/1

== matlab function sm_Experimental_Setup/Plant_PID_controlled/Non-linear Valve model/Non-linear valve ==
  data: fD input; fS input; uk input; xk output; xkp input
function xk = fcn(fD, fS, uk, xkp)
% -------------------------------------------------------------------------
% TRAINING circuit for DDPG-RL Agent | Plant Model (RLVC4 | 09-Oct-2020)
% Non-Linear valve model: Capaci and Scali (2018)
% -------------------------------------------------------------------------
% uk - fD   if uk - xk−1 > fS
% uk + fD   if uk - xk−1 < -fS
% xk - 1    if |uk - xk−1| < fS
% -------------------------------------------------------------------------
% Graded Learning Stages:
% GRADE_I    TIME_DELAY=0.1; fS = 8.4/10; fD = 3.5243/10 
% GRADE_II   TIME_DELAY=0.5; fS = 8.4/5; fD = 3.5243/5
% GRADE_III  TIME_DELAY=1.5; fS = 8.4/2; fD = 3.5243/2
% GRADE_IV   TIME_DELAY=1.5; fS = 8.4/1.5; fD = 3.5243/1.5
% GRADE_IV   TIME_DELAY=1.5, fS/1.5 and fD/1.5
% GRADE_V    TIME_DELAY=2.0, fS/1.5 and fD/1.5
% GRADE_VI   TIME_DELAY=2.5, fS/1.0 and fD/1.0
% -------------------------------------------------------------------------
    
    % For PPO, the action is a column vector [2 1], therefore we need
    %  to convert it to a [1 1]. reshape can't be used because Reshape
    %  needs to retain number of elements. Manually extract first value
    % PPO action output is (1) Mean (2) Std. Dev and therefore we need only
    % the first value
    uk = uk(1,1);
     
    t_xk = 0.0;
   
    if ((uk-xkp) > fS)
        t_xk = uk - fD;
    elseif ((uk-xkp) < -1*fS)
        t_xk = uk + fD;
    elseif (abs(uk-xkp) < fS)
        t_xk = xkp;
    end
    
xk = t_xk;

== matlab function sm_Experimental_Setup/Plant_RL_controlled/Non-linear Valve model/Non-linear valve ==
  data: fD input; fS input; uk input; xk output; xkp input
function xk = fcn(fD, fS, uk, xkp)
% -------------------------------------------------------------------------
% TRAINING circuit for DDPG-RL Agent | Plant Model (RLVC4 | 09-Oct-2020)
% Non-Linear valve model: Capaci and Scali (2018)
% -------------------------------------------------------------------------
% uk - fD   if uk - xk−1 > fS
% uk + fD   if uk - xk−1 < -fS
% xk - 1    if |uk - xk−1| < fS
% -------------------------------------------------------------------------
% Graded Learning Stages:
% GRADE_I    TIME_DELAY=0.1; fS = 8.4/10; fD = 3.5243/10 
% GRADE_II   TIME_DELAY=0.5; fS = 8.4/5; fD = 3.5243/5
% GRADE_III  TIME_DELAY=1.5; fS = 8.4/2; fD = 3.5243/2
% GRADE_IV   TIME_DELAY=1.5; fS = 8.4/1.5; fD = 3.5243/1.5
% GRADE_IV   TIME_DELAY=1.5, fS/1.5 and fD/1.5
% GRADE_V    TIME_DELAY=2.0, fS/1.5 and fD/1.5
% GRADE_VI   TIME_DELAY=2.5, fS/1.0 and fD/1.0
% -------------------------------------------------------------------------
    
    % For PPO, the action is a column vector [2 1], therefore we need
    %  to convert it to a [1 1]. reshape can't be used because Reshape
    %  needs to retain number of elements. Manually extract first value
    % PPO action output is (1) Mean (2) Std. Dev and therefore we need only
    % the first value
    uk = uk(1,1);
     
    t_xk = 0.0;
   
    if ((uk-xkp) > fS)
        t_xk = uk - fD;
    elseif ((uk-xkp) < -1*fS)
        t_xk = uk + fD;
    elseif (abs(uk-xkp) < fS)
        t_xk = xkp;
    end
    
xk = t_xk;
